simulink model "motor"  (R2025a)
settings: Solver=VariableStepAuto  StartTime=0.0  StopTime=.05  RelTol=1e-3
settings Model: Creator=cmparedesv  LastModifiedBy=cmparedesv

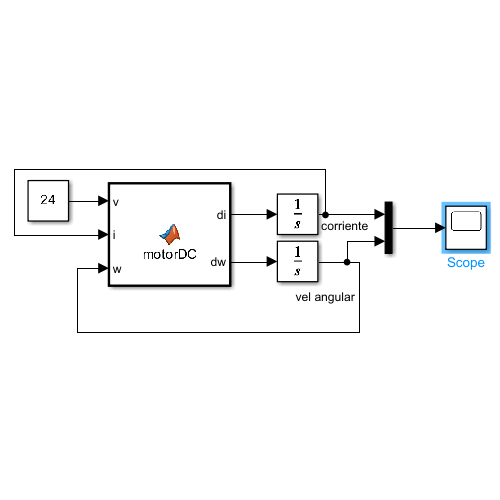
[thumbnail: Simulink's stored preview of the top-level diagram]
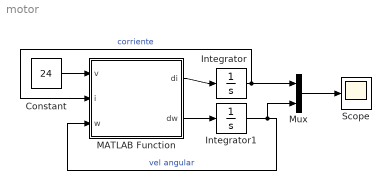
== system motor ==
  Constant : Constant  Value=24
  Integrator : Integrator
  Integrator1 : Integrator
  MATLAB Function : MATLAB Function  TreatAsAtomicUnit=on
  Mux : Mux  Inputs=2
  Scope : Scope
      settings: ActiveDisplayYMinimum=-0.299027326167429  ActiveDisplayYMaximum=2.6912459355068616
  wires:
  MATLAB Function/1(di) -> Integrator/1
  Integrator/1 -> Mux/1, MATLAB Function/2(i)  "corriente"
  MATLAB Function/2(dw) -> Integrator1/1
  Integrator1/1 -> Mux/2, MATLAB Function/3(w)  "vel angular"
  Mux/1 -> Scope/1
  Constant/1 -> MATLAB Function/1(v)

== matlab function motor/MATLAB Function ==
  data: di output; dw output; v input; i input; w input
function [di,dw] = motorDC(v,i,w)
%-----parametros----
R = 10;
L = 1e-3;
Ka = 0.5;
B = 0.8;
Km = 0.5;
J= 0.005;

%--ecuaciones---
Ea = Ka*w;
Tm = Km*i;
di = (v-R*i-Ea)/L;
dw = (Tm-B*w)/J;
